simulink model "ieee13_hif_twin_system"  (R2025a)
settings: Solver=FixedStepDiscrete  StartTime=0.0  StopTime=0.3  FixedStep=50e-6  RelTol=1e-3
model workspace (MAT data in the model file):
  BrkOpDelaySteps = 0
  InterlockEnable = 0
  InterlockMarginSteps = 1200
  Rn_arc = 300
  Rp_arc = 200
  Vn_arc = 2000
  Vp_arc = 1500
undefined symbols (not defined in the file or in its folder): D1, Delta
libraries: spsGroundLib x51, spsSeriesRLCLoadLib x39, spsSeriesRLCBranchLib x28, spsThreePhasePISectionLineLib x20, spsDiodeLib x12, spsDCVoltageSourceLib x12, spsThreePhaseBreakerLib x8, spsBreakerLib x7, spsThreePhaseVIMeasurementLib x6, spsCurrentMeasurementLib x6, spsThreePhaseSourceLib x2, spsThreePhaseTransformerTwoWindingsLib x2
(part 2 of 2)

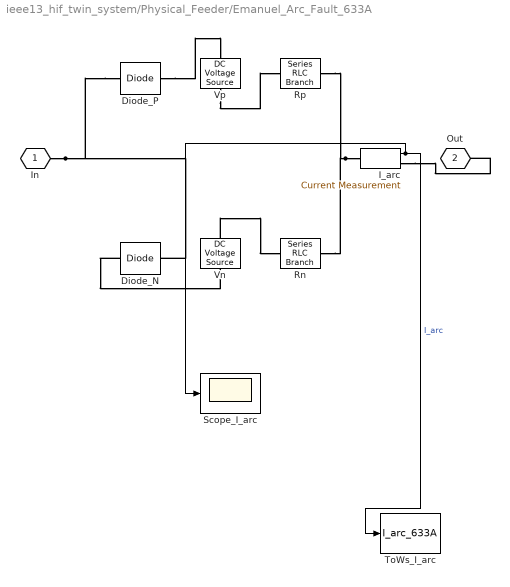
== system ieee13_hif_twin_system/Physical_Feeder/Emanuel_Arc_Fault_633A ==
  Diode_N : spsDiodeLib/Diode  Ron=0.001  Lon=0  Vf=0.8  IC=0  UseSnubber=1  Rs=1e6  Cs=inf  Measurements=off
  Diode_P : spsDiodeLib/Diode  Ron=0.001  Lon=0  Vf=0.8  IC=0  UseSnubber=1  Rs=1e6  Cs=inf  Measurements=off
  I_arc : spsCurrentMeasurementLib/Current Measurement  PhasorSimulation=off  OutputType=Complex  PSBequivalent=0
  Rn : spsSeriesRLCBranchLib/Series RLC Branch  LConnTagsString=__new0  RConnTagsString=__new0  BranchType=R  Resistance=Rn_arc  Inductance=1e-3  SetiL0=off  InitialCurrent=0  Capacitance=1e-6  Setx0=off  InitialVoltage=0  Measurements=None
  Rp : spsSeriesRLCBranchLib/Series RLC Branch  LConnTagsString=__new0  RConnTagsString=__new0  BranchType=R  Resistance=Rp_arc  Inductance=1e-3  SetiL0=off  InitialCurrent=0  Capacitance=1e-6  Setx0=off  InitialVoltage=0  Measurements=None
  Scope_I_arc : Scope
  ToWs_I_arc : ToWorkspace  VariableName=I_arc_633A  SaveFormat=Timeseries  SampleTime=-1
  Vn : spsDCVoltageSourceLib/DC Voltage Source  Amplitude=Vn_arc  Measurements=None
  Vp : spsDCVoltageSourceLib/DC Voltage Source  Amplitude=Vp_arc  Measurements=None
  In : PMIOPort  Side=Left
  Out : PMIOPort  Port=2  Side=Left
  wires:
  I_arc/1 -> Scope_I_arc/1, ToWs_I_arc/1  "I_arc"
  connections:
  Diode_P/LConn1 -- In/RConn1 -- Diode_N/RConn1
  I_arc/LConn1 -- Rp/RConn1 -- Rn/RConn1
  Diode_N/LConn1 -- Vn/LConn1
  Vn/RConn1 -- Rn/LConn1
  I_arc/RConn1 -- Out/RConn1
  Diode_P/RConn1 -- Vp/RConn1
  Vp/LConn1 -- Rp/LConn1

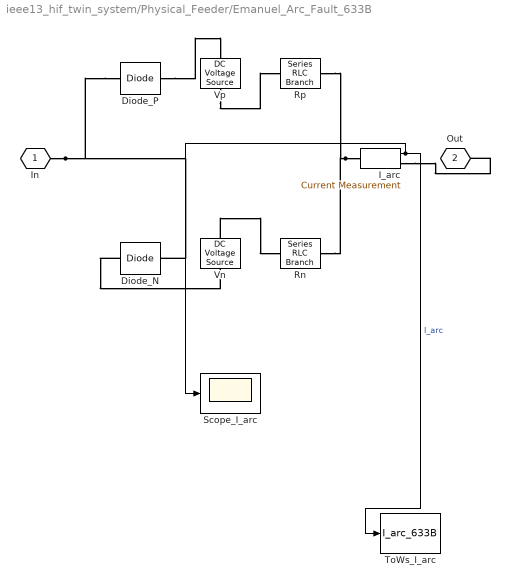
== system ieee13_hif_twin_system/Physical_Feeder/Emanuel_Arc_Fault_633B ==
  Diode_N : spsDiodeLib/Diode  Ron=0.001  Lon=0  Vf=0.8  IC=0  UseSnubber=1  Rs=1e6  Cs=inf  Measurements=off
  Diode_P : spsDiodeLib/Diode  Ron=0.001  Lon=0  Vf=0.8  IC=0  UseSnubber=1  Rs=1e6  Cs=inf  Measurements=off
  I_arc : spsCurrentMeasurementLib/Current Measurement  PhasorSimulation=off  OutputType=Complex  PSBequivalent=0
  Rn : spsSeriesRLCBranchLib/Series RLC Branch  LConnTagsString=__new0  RConnTagsString=__new0  BranchType=R  Resistance=Rn_arc  Inductance=1e-3  SetiL0=off  InitialCurrent=0  Capacitance=1e-6  Setx0=off  InitialVoltage=0  Measurements=None
  Rp : spsSeriesRLCBranchLib/Series RLC Branch  LConnTagsString=__new0  RConnTagsString=__new0  BranchType=R  Resistance=Rp_arc  Inductance=1e-3  SetiL0=off  InitialCurrent=0  Capacitance=1e-6  Setx0=off  InitialVoltage=0  Measurements=None
  Scope_I_arc : Scope
  ToWs_I_arc : ToWorkspace  VariableName=I_arc_633B  SaveFormat=Timeseries  SampleTime=-1
  Vn : spsDCVoltageSourceLib/DC Voltage Source  Amplitude=Vn_arc  Measurements=None
  Vp : spsDCVoltageSourceLib/DC Voltage Source  Amplitude=Vp_arc  Measurements=None
  In : PMIOPort  Side=Left
  Out : PMIOPort  Port=2  Side=Left
  wires:
  I_arc/1 -> Scope_I_arc/1, ToWs_I_arc/1  "I_arc"
  connections:
  Diode_P/LConn1 -- In/RConn1 -- Diode_N/RConn1
  I_arc/LConn1 -- Rp/RConn1 -- Rn/RConn1
  Diode_N/LConn1 -- Vn/LConn1
  Vn/RConn1 -- Rn/LConn1
  I_arc/RConn1 -- Out/RConn1
  Diode_P/RConn1 -- Vp/RConn1
  Vp/LConn1 -- Rp/LConn1

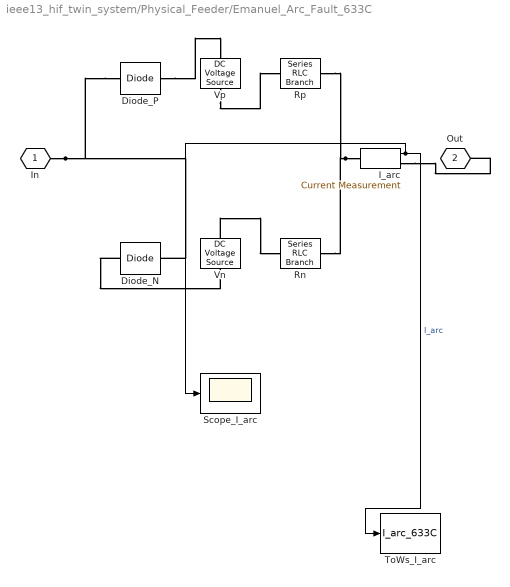
== system ieee13_hif_twin_system/Physical_Feeder/Emanuel_Arc_Fault_633C ==
  Diode_N : spsDiodeLib/Diode  Ron=0.001  Lon=0  Vf=0.8  IC=0  UseSnubber=1  Rs=1e6  Cs=inf  Measurements=off
  Diode_P : spsDiodeLib/Diode  Ron=0.001  Lon=0  Vf=0.8  IC=0  UseSnubber=1  Rs=1e6  Cs=inf  Measurements=off
  I_arc : spsCurrentMeasurementLib/Current Measurement  PhasorSimulation=off  OutputType=Complex  PSBequivalent=0
  Rn : spsSeriesRLCBranchLib/Series RLC Branch  LConnTagsString=__new0  RConnTagsString=__new0  BranchType=R  Resistance=Rn_arc  Inductance=1e-3  SetiL0=off  InitialCurrent=0  Capacitance=1e-6  Setx0=off  InitialVoltage=0  Measurements=None
  Rp : spsSeriesRLCBranchLib/Series RLC Branch  LConnTagsString=__new0  RConnTagsString=__new0  BranchType=R  Resistance=Rp_arc  Inductance=1e-3  SetiL0=off  InitialCurrent=0  Capacitance=1e-6  Setx0=off  InitialVoltage=0  Measurements=None
  Scope_I_arc : Scope
  ToWs_I_arc : ToWorkspace  VariableName=I_arc_633C  SaveFormat=Timeseries  SampleTime=-1
  Vn : spsDCVoltageSourceLib/DC Voltage Source  Amplitude=Vn_arc  Measurements=None
  Vp : spsDCVoltageSourceLib/DC Voltage Source  Amplitude=Vp_arc  Measurements=None
  In : PMIOPort  Side=Left
  Out : PMIOPort  Port=2  Side=Left
  wires:
  I_arc/1 -> Scope_I_arc/1, ToWs_I_arc/1  "I_arc"
  connections:
  Diode_P/LConn1 -- In/RConn1 -- Diode_N/RConn1
  I_arc/LConn1 -- Rp/RConn1 -- Rn/RConn1
  Diode_N/LConn1 -- Vn/LConn1
  Vn/RConn1 -- Rn/LConn1
  I_arc/RConn1 -- Out/RConn1
  Diode_P/RConn1 -- Vp/RConn1
  Vp/LConn1 -- Rp/LConn1

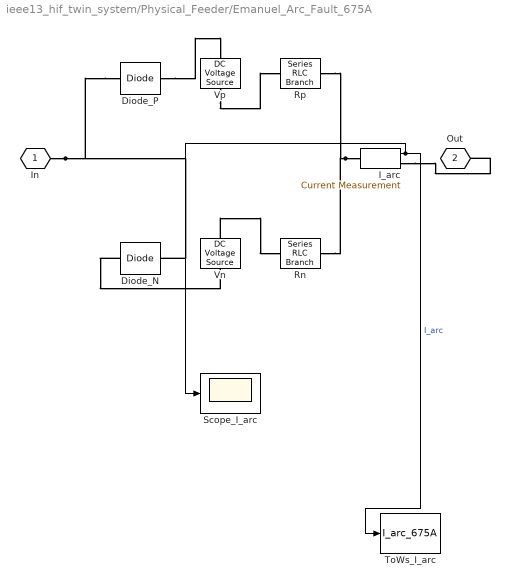
== system ieee13_hif_twin_system/Physical_Feeder/Emanuel_Arc_Fault_675A ==
  Diode_N : spsDiodeLib/Diode  Ron=0.001  Lon=0  Vf=0.8  IC=0  UseSnubber=1  Rs=1e6  Cs=inf  Measurements=off
  Diode_P : spsDiodeLib/Diode  Ron=0.001  Lon=0  Vf=0.8  IC=0  UseSnubber=1  Rs=1e6  Cs=inf  Measurements=off
  I_arc : spsCurrentMeasurementLib/Current Measurement  PhasorSimulation=off  OutputType=Complex  PSBequivalent=0
  Rn : spsSeriesRLCBranchLib/Series RLC Branch  LConnTagsString=__new0  RConnTagsString=__new0  BranchType=R  Resistance=Rn_arc  Inductance=1e-3  SetiL0=off  InitialCurrent=0  Capacitance=1e-6  Setx0=off  InitialVoltage=0  Measurements=None
  Rp : spsSeriesRLCBranchLib/Series RLC Branch  LConnTagsString=__new0  RConnTagsString=__new0  BranchType=R  Resistance=Rp_arc  Inductance=1e-3  SetiL0=off  InitialCurrent=0  Capacitance=1e-6  Setx0=off  InitialVoltage=0  Measurements=None
  Scope_I_arc : Scope
  ToWs_I_arc : ToWorkspace  VariableName=I_arc_675A  SaveFormat=Timeseries  SampleTime=-1
  Vn : spsDCVoltageSourceLib/DC Voltage Source  Amplitude=Vn_arc  Measurements=None
  Vp : spsDCVoltageSourceLib/DC Voltage Source  Amplitude=Vp_arc  Measurements=None
  In : PMIOPort  Side=Left
  Out : PMIOPort  Port=2  Side=Left
  wires:
  I_arc/1 -> Scope_I_arc/1, ToWs_I_arc/1  "I_arc"
  connections:
  Diode_P/LConn1 -- In/RConn1 -- Diode_N/RConn1
  I_arc/LConn1 -- Rp/RConn1 -- Rn/RConn1
  Diode_N/LConn1 -- Vn/LConn1
  Vn/RConn1 -- Rn/LConn1
  I_arc/RConn1 -- Out/RConn1
  Diode_P/RConn1 -- Vp/RConn1
  Vp/LConn1 -- Rp/LConn1

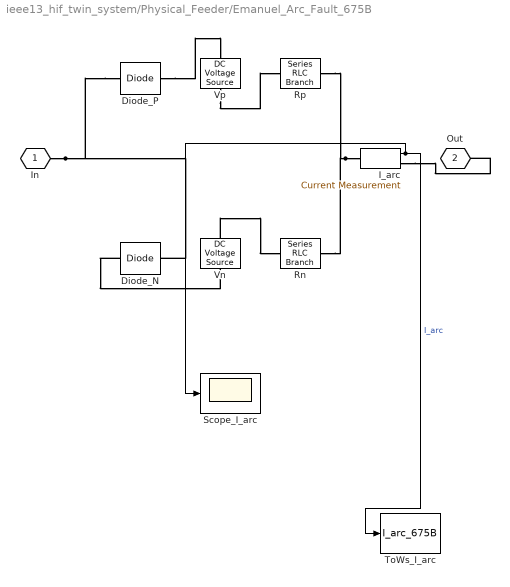
== system ieee13_hif_twin_system/Physical_Feeder/Emanuel_Arc_Fault_675B ==
  Diode_N : spsDiodeLib/Diode  Ron=0.001  Lon=0  Vf=0.8  IC=0  UseSnubber=1  Rs=1e6  Cs=inf  Measurements=off
  Diode_P : spsDiodeLib/Diode  Ron=0.001  Lon=0  Vf=0.8  IC=0  UseSnubber=1  Rs=1e6  Cs=inf  Measurements=off
  I_arc : spsCurrentMeasurementLib/Current Measurement  PhasorSimulation=off  OutputType=Complex  PSBequivalent=0
  Rn : spsSeriesRLCBranchLib/Series RLC Branch  LConnTagsString=__new0  RConnTagsString=__new0  BranchType=R  Resistance=Rn_arc  Inductance=1e-3  SetiL0=off  InitialCurrent=0  Capacitance=1e-6  Setx0=off  InitialVoltage=0  Measurements=None
  Rp : spsSeriesRLCBranchLib/Series RLC Branch  LConnTagsString=__new0  RConnTagsString=__new0  BranchType=R  Resistance=Rp_arc  Inductance=1e-3  SetiL0=off  InitialCurrent=0  Capacitance=1e-6  Setx0=off  InitialVoltage=0  Measurements=None
  Scope_I_arc : Scope
  ToWs_I_arc : ToWorkspace  VariableName=I_arc_675B  SaveFormat=Timeseries  SampleTime=-1
  Vn : spsDCVoltageSourceLib/DC Voltage Source  Amplitude=Vn_arc  Measurements=None
  Vp : spsDCVoltageSourceLib/DC Voltage Source  Amplitude=Vp_arc  Measurements=None
  In : PMIOPort  Side=Left
  Out : PMIOPort  Port=2  Side=Left
  wires:
  I_arc/1 -> Scope_I_arc/1, ToWs_I_arc/1  "I_arc"
  connections:
  Diode_P/LConn1 -- In/RConn1 -- Diode_N/RConn1
  I_arc/LConn1 -- Rp/RConn1 -- Rn/RConn1
  Diode_N/LConn1 -- Vn/LConn1
  Vn/RConn1 -- Rn/LConn1
  I_arc/RConn1 -- Out/RConn1
  Diode_P/RConn1 -- Vp/RConn1
  Vp/LConn1 -- Rp/LConn1

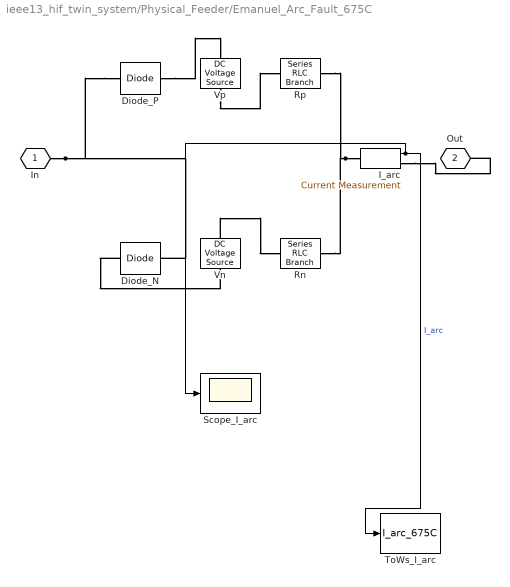
== system ieee13_hif_twin_system/Physical_Feeder/Emanuel_Arc_Fault_675C ==
  Diode_N : spsDiodeLib/Diode  Ron=0.001  Lon=0  Vf=0.8  IC=0  UseSnubber=1  Rs=1e6  Cs=inf  Measurements=off
  Diode_P : spsDiodeLib/Diode  Ron=0.001  Lon=0  Vf=0.8  IC=0  UseSnubber=1  Rs=1e6  Cs=inf  Measurements=off
  I_arc : spsCurrentMeasurementLib/Current Measurement  PhasorSimulation=off  OutputType=Complex  PSBequivalent=0
  Rn : spsSeriesRLCBranchLib/Series RLC Branch  LConnTagsString=__new0  RConnTagsString=__new0  BranchType=R  Resistance=Rn_arc  Inductance=1e-3  SetiL0=off  InitialCurrent=0  Capacitance=1e-6  Setx0=off  InitialVoltage=0  Measurements=None
  Rp : spsSeriesRLCBranchLib/Series RLC Branch  LConnTagsString=__new0  RConnTagsString=__new0  BranchType=R  Resistance=Rp_arc  Inductance=1e-3  SetiL0=off  InitialCurrent=0  Capacitance=1e-6  Setx0=off  InitialVoltage=0  Measurements=None
  Scope_I_arc : Scope
  ToWs_I_arc : ToWorkspace  VariableName=I_arc_675C  SaveFormat=Timeseries  SampleTime=-1
  Vn : spsDCVoltageSourceLib/DC Voltage Source  Amplitude=Vn_arc  Measurements=None
  Vp : spsDCVoltageSourceLib/DC Voltage Source  Amplitude=Vp_arc  Measurements=None
  In : PMIOPort  Side=Left
  Out : PMIOPort  Port=2  Side=Left
  wires:
  I_arc/1 -> Scope_I_arc/1, ToWs_I_arc/1  "I_arc"
  connections:
  Diode_P/LConn1 -- In/RConn1 -- Diode_N/RConn1
  I_arc/LConn1 -- Rp/RConn1 -- Rn/RConn1
  Diode_N/LConn1 -- Vn/LConn1
  Vn/RConn1 -- Rn/LConn1
  I_arc/RConn1 -- Out/RConn1
  Diode_P/RConn1 -- Vp/RConn1
  Vp/LConn1 -- Rp/LConn1
